simulink model "mode_v6_static_ny_initial"  (R2025b)
settings: Solver=ode45  StartTime=0.0  StopTime=10  RelTol=1e-3
model workspace (MAT data in the model file):
  A_aircraft = [-1.1  1  0; -8.558  -0.82  0; 0  1  0]
  B_aircraft = [-0.18  -1.1  0; -15.7604  -8.558  1; 0  0  0]
  C_aircraft = [0.517  0  0; 0  1  0; 0  0  1]
  D_aircraft = [0.0846  0.517  0; 0  0  0; 0  0  0]
  P.variant = 6
  P.H_km = 4
  P.V_kmh = 800
  P.Mach = 0.81
  P.V_ms = 264
  P.c1 = 0.6
  P.c2 = 8.8
  P.c3 = 15.8
  P.c4 = 1.1
  P.c5 = 0.22
  P.c6_over_g = 0.47
  P.c9 = 0.18
  P.design.static_frequency = 5
  P.design.astatic_frequency = 3
  P.design.static_pitch_outer_frequency = 0.25
  P.design.astatic_pitch_outer_frequency = 0.6
  P.design.static_ny = [-5 -5]
  P.design.astatic_ny = [-3 -3 -3]
  P.design.static_pitch = [-5 -5 -0.25]
  P.design.astatic_pitch = [-3 -3 -3 -0.6]
  P.design.result.static_ny.target = [1 10 25]
  P.design.result.static_ny.actual = [1 10 25]
  P.design.result.static_ny.desired_poles = [-5 -5]
  P.design.result.static_ny.relative_error = 1.42108547152e-16
  P.design.result.static_ny.model = 'Идеальный привод. Полная модель проверяется отдельно.'
  P.design.result.astatic_ny.target = [1 9 27 27]
  P.design.result.astatic_ny.actual = [1 9 27 27]
  P.design.result.astatic_ny.desired_poles = [-3 -3 -3]
  P.design.result.astatic_ny.relative_error = 1.31581988104e-16
  P.design.result.astatic_ny.model = 'Идеальный привод. Полная модель проверяется отдельно.'
  P.design.result.static_pitch.target = [1 10.25 27.5 6.25]
  P.design.result.static_pitch.actual = [1 10.25 27.5 6.25]
  P.design.result.static_pitch.desired_poles = [-5 -5 -0.25]
  P.design.result.static_pitch.relative_error = 6.459479416e-17
  P.design.result.static_pitch.model = 'Идеальный привод. Полная модель проверяется отдельно.'
  P.design.result.astatic_pitch.target = [1 9.6 32.4 43.2 16.2]
  P.design.result.astatic_pitch.actual = [1 9.6 32.4 43.2 16.2]
  P.design.result.astatic_pitch.desired_poles = [-3 -3 -3 -0.6]
  P.design.result.astatic_pitch.relative_error = 4.11193712824e-17
  P.design.result.astatic_pitch.model = 'Идеальный привод. Полная модель проверяется отдельно.'
  P.static.Kn = 0.849443153507
  P.static.Kw = 0.470819183687
  P.static.Ki = 0
  P.static.Ktheta = 0
  P.astatic.Kn = 1.1529355114
  P.astatic.Kw = 0.416220354446
  P.astatic.Ki = 3.28206773394
  P.pitch_static.Kn = 0.410194974021
  P.pitch_static.Kw = 0.5077761652
  P.pitch_static.Ktheta = 0.931115896549
  P.pitch_astatic.Kn = 1.6128495192
  P.pitch_astatic.Kw = 0.428164626752
  P.pitch_astatic.Ki = 3.14481149083
  P.pitch_astatic.Ktheta = 0.281619182974
  P.f1 = 1.92
  P.f0 = 9.46
  P.omega_aircraft = 3.07571129985
  P.zeta_aircraft = 0.312122922606
  P.actuator.dynamic = 1
  P.actuator.Omega = 30
  P.actuator.zeta = 0.8
  P.actuator.options = [5 10 15 20 25 30]
  P.reference.static_ny.Kn = 1.11
  P.reference.static_ny.Kw = 0.32
  P.reference.static_ny.Ki = 0
  P.reference.static_ny.Ktheta = 0
  P.reference.astatic_ny.Kn = 1.16
  P.reference.astatic_ny.Kw = 0.44
  P.reference.astatic_ny.Ki = 5.25
  P.reference.astatic_ny.Ktheta = 0
  P.reference.static_pitch.Kn = 1.11
  P.reference.static_pitch.Kw = 0.32
  P.reference.static_pitch.Ki = 0
  P.reference.static_pitch.Ktheta = 1
  P.reference.astatic_pitch.Kn = 1.16
  P.reference.astatic_pitch.Kw = 0.44
  P.reference.astatic_pitch.Ki = 5.25
  P.reference.astatic_pitch.Ktheta = 0.3
  P.refinement.max_iterations = 200
  P.refinement.max_evaluations = 1000
  P.refinement.max_seconds = 60
  P.refinement.max_overshoot = 10
  P.refinement.target_time = 1
  P.refinement.band = 0.05
  P.refinement.dt = 0.01
  P.refinement.validation_dt = 0.002
  P.refinement.horizon = 30
  P.refinement.lower = [0.001 0.001 0.001 0.001]
  P.refinement.upper = [15 8 40 8]
  P.t_end = 10
  P.dt = 0.01
  P.command.ny = 1
  P.command.theta = 1
  P.command.gust = 1
  P.command.moment = 1
  P.sweep.c2 = [0.5 1 1.5]
  P.sweep.c1 = [0.5 1 1.5]
  P.sweep.c9 = [0 1 2]
  P.sweep.Omega = [0.5 1 2]
  P.sweep.Kw = [0.5 1 1.5]
  P.sweep.Kn = [0.5 1 1.5]
  P.sweep.Ktheta = [0.5 1 1.5]
settings Model: Creator=egorbelozercev  LastModifiedBy=egorbelozercev

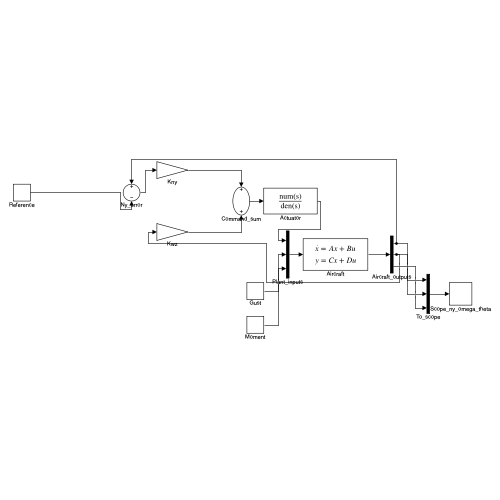
[thumbnail: Simulink's stored preview of the top-level diagram]
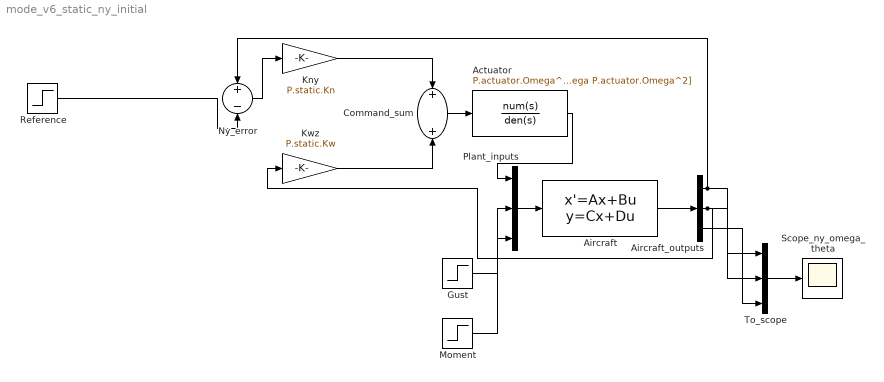
== system mode_v6_static_ny_initial ==
  Actuator : TransferFcn  Numerator=P.actuator.Omega^2  Denominator=[1 2*P.actuator.zeta*P.actuator.Omega P.actuator.Omega^2]
  Aircraft : StateSpace  A=A_aircraft  B=B_aircraft  C=C_aircraft  D=D_aircraft  InitialCondition=0
  Aircraft_outputs : Demux  Outputs=3
  Command_sum : Sum
  Gust : Step  Time=0  After=0  SampleTime=0
  Kny : Gain  Gain=P.static.Kn
  Kwz : Gain  Gain=P.static.Kw
  Moment : Step  Time=0  After=0  SampleTime=0
  Ny_error : Sum  Inputs=+-
  Plant_inputs : Mux  Inputs=3
  Reference : Step  Time=0  SampleTime=0
  Scope_ny_omega_theta : Scope
  To_scope : Mux  Inputs=3
  wires:
  Reference/1 -> Ny_error/2
  Ny_error/1 -> Kny/1
  Aircraft_outputs/1 -> Ny_error/1, To_scope/1
  Aircraft_outputs/2 -> Kwz/1, To_scope/2
  Kny/1 -> Command_sum/1
  Kwz/1 -> Command_sum/2
  Command_sum/1 -> Actuator/1
  Actuator/1 -> Plant_inputs/1
  Gust/1 -> Plant_inputs/2
  Moment/1 -> Plant_inputs/3
  Plant_inputs/1 -> Aircraft/1
  Aircraft/1 -> Aircraft_outputs/1
  Aircraft_outputs/3 -> To_scope/3
  To_scope/1 -> Scope_ny_omega_theta/1
